simulink model "cp6_ej5"  (R2026a)
settings: Solver=VariableStepAuto  StopTime=800  MaxStep=0.1
libraries: slpidlib x1
settings Model: Creator=benja  LastModifiedBy=benja

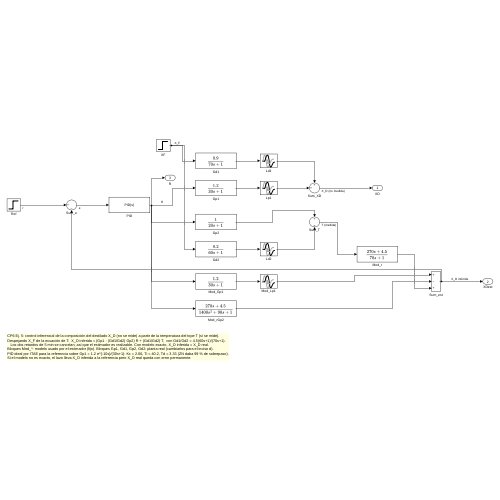
[thumbnail: Simulink's stored preview of the top-level diagram]
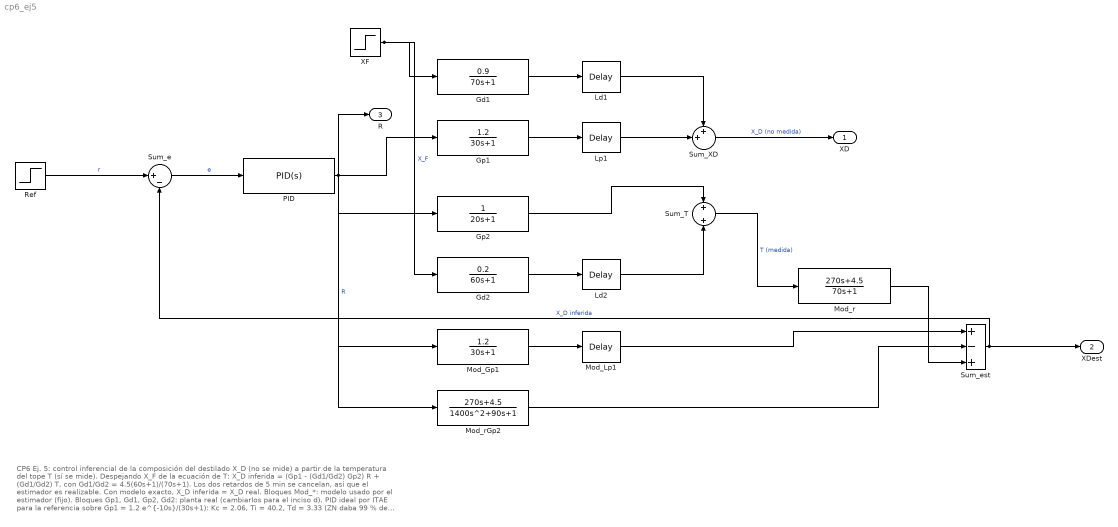
== system cp6_ej5 ==
  note: CP6 Ej. 5: control inferencial de la composición del destilado X_D (no se mide) a partir de la temperatura del tope T (sí se mide).
      | Despejando X_F de la ecuación de T:  X_D inferida = (Gp1 - (Gd1/Gd2) Gp2) R + (Gd1/Gd2) T,  con Gd1/Gd2 = 4.5(60s+1)/(70s+1).
      |    Los dos retardos de 5 min se cancelan, así que el estimador es realizable. Con modelo exacto, X_D inferida = X_D real.
      | Bloques Mod_*: modelo usado por el estimador (fijo). Bloques Gp1, Gd1, Gp2, Gd2: planta real (cambiarlos para el inciso d).
      | PID ideal por ITAE para la referencia sobre Gp1 = 1.2 e^{-10s}/(30s+1): Kc = 2.06, Ti = 40.2, Td = 3.33 (ZN daba 99 % de sobrepaso).
      | Si el modelo no es exacto, el lazo lleva X_D inferida a la referencia pero X_D real queda con error permanente.
  Gd1 : TransferFcn  Numerator=0.9  Denominator=[70 1]
  Gd2 : TransferFcn  Numerator=0.2  Denominator=[60 1]
  Gp1 : TransferFcn  Numerator=1.2  Denominator=[30 1]
  Gp2 : TransferFcn  Numerator=1  Denominator=[20 1]
  Ld1 : TransportDelay  DelayTime=5
  Ld2 : TransportDelay  DelayTime=5
  Lp1 : TransportDelay  DelayTime=10
  Mod_Gp1 : TransferFcn  Numerator=1.2  Denominator=[30 1]
  Mod_Lp1 : TransportDelay  DelayTime=10
  Mod_r : TransferFcn  Numerator=[270 4.5]  Denominator=[70 1]
  Mod_rGp2 : TransferFcn  Numerator=[270 4.5]  Denominator=[1400 90 1]
  PID : slpidlib/PID Controller  Controller=PID  Form=Ideal  TimeDomain=Continuous-time  UseExternalTs=off  SampleTime=-1  IntegratorMethod=Forward Euler  FilterMethod=Forward Euler  ControllerParametersSource=internal  P=2.0572  I=0.02490  UseKiTs=off  D=3.3299  UseExternalDerivativeSource=off  N=3.0031  UseFilter=on  TunerSelectOption=Transfer Function Based (PID Tuner App)  InitialConditionSource=internal  InitialConditionForIntegrator=0  InitialConditionForFilter=0  DifferentiatorICPrevScaledInput=0  ExternalReset=none  TrackingMode=off  Kt=1  LimitOutput=off  SatLimitsSource=internal  UpperSaturationLimit=inf  LowerSaturationLimit=-inf  LinearizeAsGain=on  AntiWindupMode=none  Kb=1  LimitIntegrator=off  UpperIntegratorSaturationLimit=inf  LowerIntegratorSaturationLimit=-inf  POutMin=[]  POutMax=[]  IOutMin=[]  IOutMax=[]  DOutMin=[]  DOutMax=[]  NOutMin=[]  NOutMax=[]  SumOutMin=[]  SumOutMax=[]  SaturationOutMin=[]  SaturationOutMax=[]  PParamMin=[]  PParamMax=[]  IParamMin=[]  IParamMax=[]  DParamMin=[]  DParamMax=[]  NParamMin=[]  NParamMax=[]  KbParamMin=[]  KbParamMax=[]  KtParamMin=[]  KtParamMax=[]  KbOutMin=[]  KbOutMax=[]  KtOutMin=[]  KtOutMax=[]  IntegratorOutMin=[]  IntegratorOutMax=[]  FilterOutMin=[]  FilterOutMax=[]  SumI1OutMin=[]  SumI1OutMax=[]  SumI2OutMin=[]  SumI2OutMax=[]  SumI3OutMin=[]  SumI3OutMax=[]  SumI4OutMin=[]  SumI4OutMax=[]  SumDOutMin=[]  SumDOutMax=[]  DifferentiatorOutMin=[]  DifferentiatorOutMax=[]  FilterDiffOutCoefMin=[]  FilterDiffOutCoefMax=[]  ReciprocalOutMin=[]  ReciprocalOutMax=[]  SumDenOutMin=[]  SumDenOutMax=[]  SumNumOutMin=[]  SumNumOutMax=[]  DivideOutMin=[]  DivideOutMax=[]  UdiffTsProdOutMin=[]  UdiffTsProdOutMax=[]  NTsProdOutMin=[]  NTsProdOutMax=[]  UintegralTsProdOutMin=[]  UintegralTsProdOutMax=[]  UngainTsProdOutMin=[]  UngainTsProdOutMax=[]  ClampingZeroOutDataTypeStr=Inherit: Inherit via back propagation  ClampingZeroOutMin=[]  ClampingZeroOutMax=[]  FilterDenConstantOutDataTypeStr=Inherit: Inherit via back propagation  FilterDenConstantOutMin=[]  FilterDenConstantOutMax=[]  PCopyOutDataTypeStr=Inherit: Inherit via back propagation  PCopyOutMin=[]  PCopyOutMax=[]  NCopyOutDataTypeStr=Inherit: Inherit via back propagation  NCopyOutMin=[]  NCopyOutMax=[]  IntegratorContinuousStateAttributes=''  IntegratorStateMustResolveToSignalObject=off  IntegratorRTWStateStorageClass=Auto  FilterContinuousStateAttributes=''  FilterStateMustResolveToSignalObject=off  FilterRTWStateStorageClass=Auto  ParallelPVariant=Passthrough  IdealPVariant=InternalParameters  IVariant=InternalParameters  DVariant=InternalParameters  IntegratorVariant=Continuous  SatVariant=Disabled  AWVariant=Passthrough  PCopyVariant=Disabled  TRVariant=Disabled  FdbkBlocksVariant=Forward  IdealPFdbkVariant=Disabled  SatFdbkVariant=Disabled  DerivativeFilterVariant=ContFilter  NVariant=InternalParameters  NCopyVariant=Disabled  FilterICVariant=InternalICsFilter  IntegratorICVariant=InternalICs  ExternalResetVariant=Disabled  TRSumVariant=Passthrough  SumFdbkVariant=Disabled  SumVariant=Sum_PID  TsampFilterVariant=InternalTs  TsampNgainVariant=Passthrough  TsampIntegralVariant=Disabled_SignalSpec  ExternalSaturationOutDataTypeStr=Inherit: Same as second input  DerivativeSourceVariant=ErrorSignal  PreIntVariant=InternalPreInt
  Ref : Step  Time=10  SampleTime=0
  Sum_T : Sum  Inputs=+|+
  Sum_XD : Sum  Inputs=++|
  Sum_e : Sum  Inputs=|+-
  Sum_est : Sum  Inputs=+-+
  XF : Step  Time=400  SampleTime=0
  XD : Outport
  XDest : Outport  Port=2
  R : Outport  Port=3
  wires:
  Ref/1 -> Sum_e/1  "r"
  Sum_e/1 -> PID/1  "e"
  PID/1 -> Gp1/1, Gp2/1, Mod_Gp1/1, Mod_rGp2/1, R/1  "R"
  Gp1/1 -> Lp1/1
  Lp1/1 -> Sum_XD/2
  XF/1 -> Gd1/1, Gd2/1  "X_F"
  Gd1/1 -> Ld1/1
  Ld1/1 -> Sum_XD/1
  Sum_XD/1 -> XD/1  "X_D (no medida)"
  Gp2/1 -> Sum_T/1
  Gd2/1 -> Ld2/1
  Ld2/1 -> Sum_T/2
  Mod_Gp1/1 -> Mod_Lp1/1
  Mod_Lp1/1 -> Sum_est/1
  Mod_rGp2/1 -> Sum_est/2
  Sum_T/1 -> Mod_r/1  "T (medida)"
  Mod_r/1 -> Sum_est/3
  Sum_est/1 -> XDest/1, Sum_e/2  "X_D inferida"
